simulink model "ids_sim_harness"  (R2024a)
settings: Solver=FixedStepDiscrete  StartTime=0.0  StopTime=130  FixedStep=0.1  RelTol=1e-3
model workspace (MAT data in the model file):
  A_btnAck = [0 0.1 0.2 0.3 0.4 0.5 0.6 0.7 0.8 0.9 1 1.1 ... (2602 elements, 1301x2)]
  A_btnArm = [0 0.1 0.2 0.3 0.4 0.5 0.6 0.7 0.8 0.9 1 1.1 ... (2602 elements, 1301x2)]
  A_btnSiren = [0 0.1 0.2 0.3 0.4 0.5 0.6 0.7 0.8 0.9 1 1.1 ... (2602 elements, 1301x2)]
  A_gps = [0 0.1 0.2 0.3 0.4 0.5 0.6 0.7 0.8 0.9 1 1.1 ... (5204 elements, 1301x4)]
  A_gyro = [0 0.1 0.2 0.3 0.4 0.5 0.6 0.7 0.8 0.9 1 1.1 ... (5204 elements, 1301x4)]
  A_lux = [0 0.1 0.2 0.3 0.4 0.5 0.6 0.7 0.8 0.9 1 1.1 ... (2602 elements, 1301x2)]
  A_ori = [0 0.1 0.2 0.3 0.4 0.5 0.6 0.7 0.8 0.9 1 1.1 ... (5204 elements, 1301x4)]
  A_role = [0 0.1 0.2 0.3 0.4 0.5 0.6 0.7 0.8 0.9 1 1.1 ... (2602 elements, 1301x2)]
  B_btnAck = [0 0.1 0.2 0.3 0.4 0.5 0.6 0.7 0.8 0.9 1 1.1 ... (2602 elements, 1301x2)]
  B_btnArm = [0 0.1 0.2 0.3 0.4 0.5 0.6 0.7 0.8 0.9 1 1.1 ... (2602 elements, 1301x2)]
  B_btnSiren = [0 0.1 0.2 0.3 0.4 0.5 0.6 0.7 0.8 0.9 1 1.1 ... (2602 elements, 1301x2)]
  B_gps = [0 0.1 0.2 0.3 0.4 0.5 0.6 0.7 0.8 0.9 1 1.1 ... (5204 elements, 1301x4)]
  B_gyro = [0 0.1 0.2 0.3 0.4 0.5 0.6 0.7 0.8 0.9 1 1.1 ... (5204 elements, 1301x4)]
  B_lux = [0 0.1 0.2 0.3 0.4 0.5 0.6 0.7 0.8 0.9 1 1.1 ... (2602 elements, 1301x2)]
  B_ori = [0 0.1 0.2 0.3 0.4 0.5 0.6 0.7 0.8 0.9 1 1.1 ... (5204 elements, 1301x4)]
  B_role = [0 0.1 0.2 0.3 0.4 0.5 0.6 0.7 0.8 0.9 1 1.1 ... (2602 elements, 1301x2)]
(part 1 of 2)
settings Model: Creator=prana  LastModifiedBy=prana

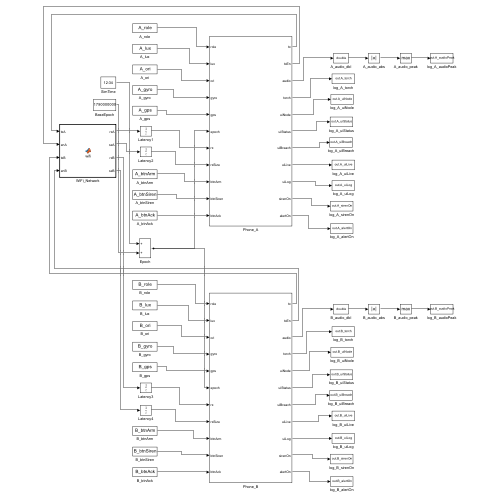
[thumbnail: Simulink's stored preview of the top-level diagram]
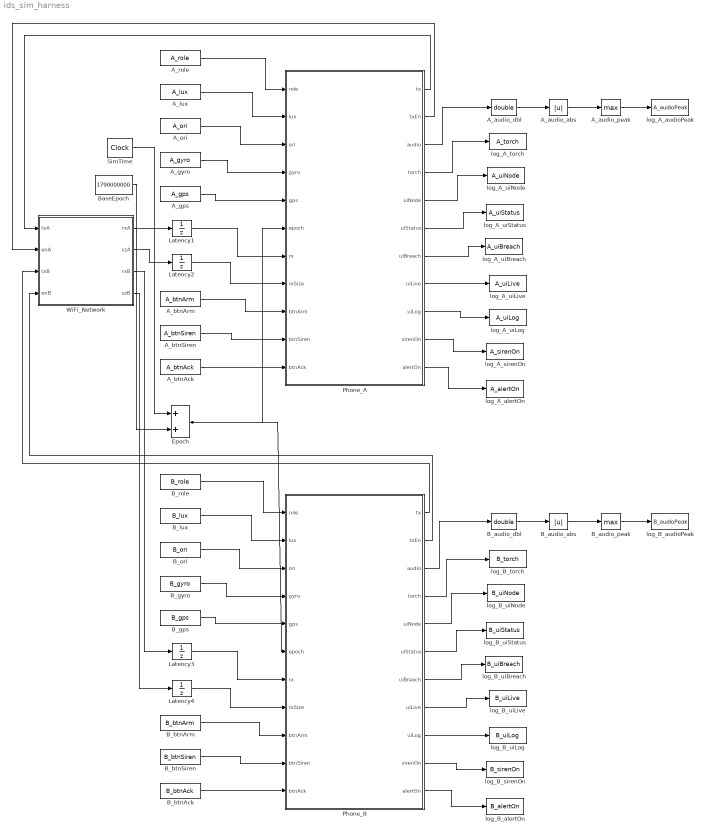
== system ids_sim_harness ==
  A_audio_abs : Abs  SaturateOnIntegerOverflow=off
  A_audio_dbl : DataTypeConversion  OutDataTypeStr=double  SaturateOnIntegerOverflow=off  RndMeth=Floor
  A_audio_peak : MinMax  Function=max
  A_btnAck : FromWorkspace  VariableName=A_btnAck  SampleTime=0.1  Interpolate=off  OutputAfterFinalValue=Holding final value
  A_btnArm : FromWorkspace  VariableName=A_btnArm  SampleTime=0.1  Interpolate=off  OutputAfterFinalValue=Holding final value
  A_btnSiren : FromWorkspace  VariableName=A_btnSiren  SampleTime=0.1  Interpolate=off  OutputAfterFinalValue=Holding final value
  A_gps : FromWorkspace  VariableName=A_gps  SampleTime=0.1  Interpolate=off  OutputAfterFinalValue=Holding final value
  A_gyro : FromWorkspace  VariableName=A_gyro  SampleTime=0.1  Interpolate=off  OutputAfterFinalValue=Holding final value
  A_lux : FromWorkspace  VariableName=A_lux  SampleTime=0.1  Interpolate=off  OutputAfterFinalValue=Holding final value
  A_ori : FromWorkspace  VariableName=A_ori  SampleTime=0.1  Interpolate=off  OutputAfterFinalValue=Holding final value
  A_role : FromWorkspace  VariableName=A_role  SampleTime=0.1  Interpolate=off  OutputAfterFinalValue=Holding final value
  B_audio_abs : Abs  SaturateOnIntegerOverflow=off
  B_audio_dbl : DataTypeConversion  OutDataTypeStr=double  SaturateOnIntegerOverflow=off  RndMeth=Floor
  B_audio_peak : MinMax  Function=max
  B_btnAck : FromWorkspace  VariableName=B_btnAck  SampleTime=0.1  Interpolate=off  OutputAfterFinalValue=Holding final value
  B_btnArm : FromWorkspace  VariableName=B_btnArm  SampleTime=0.1  Interpolate=off  OutputAfterFinalValue=Holding final value
  B_btnSiren : FromWorkspace  VariableName=B_btnSiren  SampleTime=0.1  Interpolate=off  OutputAfterFinalValue=Holding final value
  B_gps : FromWorkspace  VariableName=B_gps  SampleTime=0.1  Interpolate=off  OutputAfterFinalValue=Holding final value
  B_gyro : FromWorkspace  VariableName=B_gyro  SampleTime=0.1  Interpolate=off  OutputAfterFinalValue=Holding final value
  B_lux : FromWorkspace  VariableName=B_lux  SampleTime=0.1  Interpolate=off  OutputAfterFinalValue=Holding final value
  B_ori : FromWorkspace  VariableName=B_ori  SampleTime=0.1  Interpolate=off  OutputAfterFinalValue=Holding final value
  B_role : FromWorkspace  VariableName=B_role  SampleTime=0.1  Interpolate=off  OutputAfterFinalValue=Holding final value
  BaseEpoch : Constant  Value=1790000000
  Epoch : Sum
  Latency{1..4} (4 alike) : UnitDelay  SampleTime=0.1  HasFrameUpgradeWarning=on
  Phone_A : Subsystem
  Phone_B : Subsystem
  SimTime : DigitalClock  SampleTime=0.1
  WiFi_Network : MATLAB Function  TreatAsAtomicUnit=on
  log_A_alertOn : ToWorkspace  VariableName=A_alertOn  SampleTime=-1
  log_A_audioPeak : ToWorkspace  VariableName=A_audioPeak  SampleTime=-1
  log_A_sirenOn : ToWorkspace  VariableName=A_sirenOn  SampleTime=-1
  log_A_torch : ToWorkspace  VariableName=A_torch  SampleTime=-1
  log_A_uiBreach : ToWorkspace  VariableName=A_uiBreach  SampleTime=-1
  log_A_uiLive : ToWorkspace  VariableName=A_uiLive  SampleTime=-1
  log_A_uiLog : ToWorkspace  VariableName=A_uiLog  SampleTime=-1
  log_A_uiNode : ToWorkspace  VariableName=A_uiNode  SampleTime=-1
  log_A_uiStatus : ToWorkspace  VariableName=A_uiStatus  SampleTime=-1
  log_B_alertOn : ToWorkspace  VariableName=B_alertOn  SampleTime=-1
  log_B_audioPeak : ToWorkspace  VariableName=B_audioPeak  SampleTime=-1
  log_B_sirenOn : ToWorkspace  VariableName=B_sirenOn  SampleTime=-1
  log_B_torch : ToWorkspace  VariableName=B_torch  SampleTime=-1
  log_B_uiBreach : ToWorkspace  VariableName=B_uiBreach  SampleTime=-1
  log_B_uiLive : ToWorkspace  VariableName=B_uiLive  SampleTime=-1
  log_B_uiLog : ToWorkspace  VariableName=B_uiLog  SampleTime=-1
  log_B_uiNode : ToWorkspace  VariableName=B_uiNode  SampleTime=-1
  log_B_uiStatus : ToWorkspace  VariableName=B_uiStatus  SampleTime=-1
  wires:
  SimTime/1 -> Epoch/1
  BaseEpoch/1 -> Epoch/2
  A_audio_abs/1 -> A_audio_peak/1
  Phone_A/1(tx) -> WiFi_Network/1(txA)
  WiFi_Network/1(rxA) -> Latency1/1
  WiFi_Network/4(szB) -> Latency4/1
  Phone_B/6(uiStatus) -> log_B_uiStatus/1
  WiFi_Network/3(rxB) -> Latency3/1
  Phone_B/4(torch) -> log_B_torch/1
  WiFi_Network/2(szA) -> Latency2/1
  A_lux/1 -> Phone_A/2(lux)
  A_role/1 -> Phone_A/1(role)
  A_ori/1 -> Phone_A/3(ori)
  A_gyro/1 -> Phone_A/4(gyro)
  A_audio_dbl/1 -> A_audio_abs/1
  A_gps/1 -> Phone_A/5(gps)
  Phone_B/10(sirenOn) -> log_B_sirenOn/1
  Latency3/1 -> Phone_B/7(rx)
  Latency2/1 -> Phone_A/8(rxSize)
  Latency1/1 -> Phone_A/7(rx)
  A_btnArm/1 -> Phone_A/9(btnArm)
  A_btnSiren/1 -> Phone_A/10(btnSiren)
  A_btnAck/1 -> Phone_A/11(btnAck)
  B_role/1 -> Phone_B/1(role)
  Epoch/1 -> Phone_B/6(epoch), Phone_A/6(epoch)
  Phone_A/5(uiNode) -> log_A_uiNode/1
  B_lux/1 -> Phone_B/2(lux)
  B_ori/1 -> Phone_B/3(ori)
  Phone_A/2(txEn) -> WiFi_Network/2(enA)
  B_gyro/1 -> Phone_B/4(gyro)
  B_gps/1 -> Phone_B/5(gps)
  B_btnSiren/1 -> Phone_B/10(btnSiren)
  Latency4/1 -> Phone_B/8(rxSize)
  A_audio_peak/1 -> log_A_audioPeak/1
  Phone_A/3(audio) -> A_audio_dbl/1
  B_btnArm/1 -> Phone_B/9(btnArm)
  Phone_A/8(uiLive) -> log_A_uiLive/1
  B_btnAck/1 -> Phone_B/11(btnAck)
  B_audio_peak/1 -> log_B_audioPeak/1
  Phone_A/4(torch) -> log_A_torch/1
  Phone_A/6(uiStatus) -> log_A_uiStatus/1
  B_audio_dbl/1 -> B_audio_abs/1
  Phone_A/7(uiBreach) -> log_A_uiBreach/1
  Phone_A/9(uiLog) -> log_A_uiLog/1
  Phone_A/10(sirenOn) -> log_A_sirenOn/1
  Phone_A/11(alertOn) -> log_A_alertOn/1
  Phone_B/1(tx) -> WiFi_Network/3(txB)
  Phone_B/2(txEn) -> WiFi_Network/4(enB)
  Phone_B/3(audio) -> B_audio_dbl/1
  Phone_B/5(uiNode) -> log_B_uiNode/1
  Phone_B/7(uiBreach) -> log_B_uiBreach/1
  Phone_B/8(uiLive) -> log_B_uiLive/1
  Phone_B/9(uiLog) -> log_B_uiLog/1
  Phone_B/11(alertOn) -> log_B_alertOn/1
  B_audio_abs/1 -> B_audio_peak/1
